simulink model "Mission_Server_Swarm_2QDrone"  (Simulink 9.1)
settings: Solver=ode2  StartTime=0.0  StopTime=inf  FixedStep=0.001  RelTol=1e-3  EnableMultiTasking=on
undefined symbols (not defined in the file): Host, qc_get_step_size
libraries: quarc_library x31, simulink x8
(part 1 of 2)
settings Model: Creator=Admin  LastModifiedBy=jpineros  SimulationMode=external  ExtModeTrigDuration=10000
settings SolverCC: PositivePriorityOrder=on
settings DataIOCC: SaveFormat=Dataset
settings OptimizationCC: LifeSpan=auto
settings DebuggingCC: UnderspecifiedInitializationDetection=Simplified  MergeDetectMultiDrivingBlocksExec=error
settings HardwareCC: ProdBitPerPointer=64  ProdBitPerSizeT=64  ProdBitPerPtrDiffT=64  ProdLargestAtomicFloat=Float  ProdIntDivRoundTo=Zero  ProdEndianess=LittleEndian  ProdWordSize=64  ProdHWDeviceType=Intel->x86-64 (Windows64)
settings ModelReferenceCC: PropagateSignalLabelsOutOfModel=on
settings RTWCC: SystemTargetFile=quarc_win64.tlc  TemplateMakefile=quarc_default_tmf  Description=QUARC Win64 Target Using Toolchain  Toolchain=QUARC win64 | nmake (64-bit Windows)  BuildConfiguration=Faster Runs
settings STFCustomTargetCC: ConcurrentExecutionCompliant=on  UseToolchainInfoCompliant=on  SystemTargetFile=quarc_win64.tlc
settings GRTTargetCC: ParMdlRefBuildCompliant=off  CompOptLevelCompliant=off  MatFileLogging=off  CPPClassGenCompliant=off  ExtMode=on  ExtModeMexFile=quarc_comm
settings ConfigComp: CovHtmlReporting=off

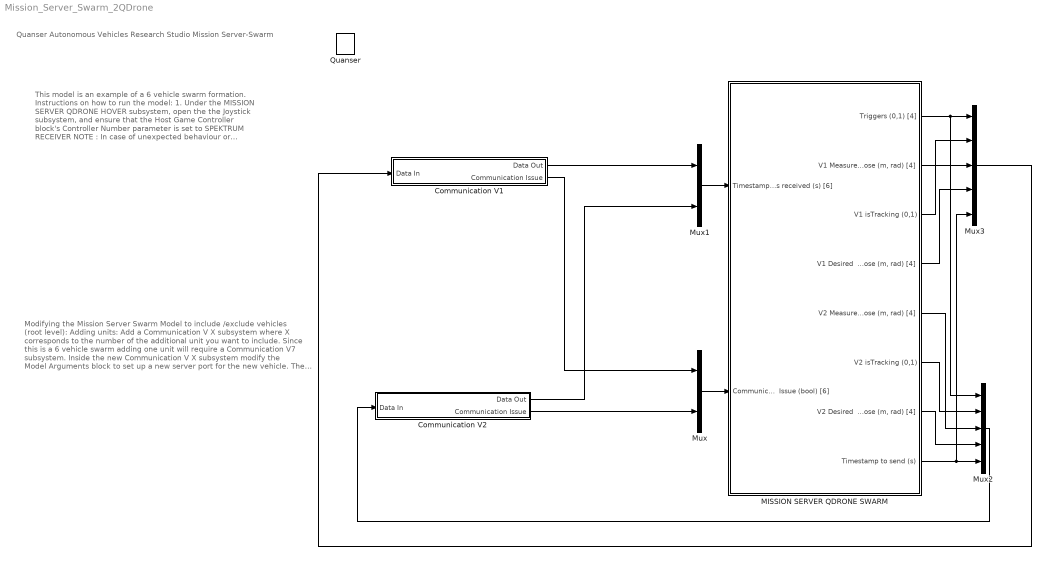
== system Mission_Server_Swarm_2QDrone ==
  note: Modifying the Mission Server Swarm Model to include /exclude vehicles (root level):
      |
      | Adding units:
      | Add a Communication V X subsystem where X corresponds to the number of the additional unit you want to include. Since this is a 6 vehicle swarm adding one unit will require a Communication V7 subsystem.
      | Inside the new Communication V X subsystem modify the Model Arguments block to set up a new server port for the new vehicle. The convention for the Model arguments is URI_Host_V X , where X corresponds to the number of the additional unit you want to include.
      | Go to Simulation\Model Configuration Parameters\Code Generation\Interface in here modify the MEX-File Arguments to include the new Model Argument defined in step 2. This is also where the new port number related to the new vehicle needs to be defined. The format for this new argument should be -URI_Host_VX tcpip://localhost:1800X and must be included within the identifiers ' ' . An example of a modied MEX-Files Arguments string for a 7 vehicle case looks as follows: '-w -d %d -uri %u -URI_Host_V1 tcpip://localhost:18001 -URI_Host_V2 tcpip://localhost:18002 -URI_Host_V3 tcpip://localhost:18003 -URI_Host_V4 tcpip://localhost:18004 -URI_Host_V5 tcpip://localhost:18005 -URI_Host_V6 tcpip://localhost:18006 -URI_Host_V7 tcpip://localhost:18007'
      | Go inside the MISSION SERVER QDRONE SWARM subsystem and follow the instructions on how to add additional units.
      |
      | Removing Units:
      | Remove the excess number of Communication VX subsystems.
      | Go to Simulation\Model Configuration Parameters\Code Generation\Interface in here modify the MEX-File Arguments to match the new number of Communication VX subsystems that you would like to use. An example of a modifified MEX-File Arguments string for a 3 vehicle case looks as follows: '-w -d %d -uri %u -URI_Host_V1 tcpip://localhost:18001 -URI_Host_V2 tcpip://localhost:18002 -URI_Host_V3 tcpip://localhost:18003'
      | Go inside the MISSION SERVER QDRONE SWARM subsystem and follow the instructions on how to remove the number of excess units.
  note: This model is an example of a 6 vehicle swarm formation.
      |
      | Instructions on how to run the model:
      |
      | 1. Under the MISSION SERVER QDRONE HOVER subsystem, open the the Joystick subsystem, and ensure that the Host Game Controller block's Controller Number parameter is set to SPEKTRUM RECEIVER
      | NOTE : In case of unexpected behaviour or emergencies, use the Emergency Abort to cut all power to the motors (this will result in the drone falling). This
      | 2. Configure the localization information for the 6 agents in the Data Server (Localization) subsystem.
      | 3. Under the QUARC menu, click on Build .
      | 4. Under the QUARC menu, click on Start . Wait for the model to start running.
      | 5. Ensure that the isTracking? display shows 1 and that the Joystick Issue display shows 0 (joystick must be powered ON with USB dongle attached to the PC).
      |
      | NOTE : At the start of the model the Comm Issue with Commander display SHOULD display 0. Once the Commander_Stabilizer has successfully connected to the mission server the communication issue flag will update. Landing the QDrones will stop the Commander_Stabilizer model at which point the Comm Issue with Commander should show 1. To close the warning window please stop the Mission_Server_Swarm model.
  note: Quanser Autonomous Vehicles Research Studio
      | Mission Server-Swarm
  Communication V1 : Subsystem
  Communication V2 : Subsystem
  MISSION SERVER QDRONE SWARM : Subsystem
  Mux : Mux  Inputs=2
  Mux1 : Mux  Inputs=2
  Mux2 : Mux  Inputs=5
  Mux3 : Mux  Inputs=5
  Quanser : quarc_library/Logos/Quanser
  wires:
  Mux/1 -> MISSION SERVER QDRONE SWARM/2(Communication  Issue (bool) [6])
  Mux1/1 -> MISSION SERVER QDRONE SWARM/1(Timestamps received (s) [6])
  MISSION SERVER QDRONE SWARM/3(V1 isTracking (0,1)) -> Mux3/2
  MISSION SERVER QDRONE SWARM/1(Triggers (0,1) [4]) -> Mux2/1, Mux3/1
  MISSION SERVER QDRONE SWARM/4("V1 Desired  Pose (m, rad) [4]") -> Mux3/4
  Mux3/1 -> Communication V1/1(Data In)
  Mux2/1 -> Communication V2/1(Data In)
  MISSION SERVER QDRONE SWARM/2("V1 Measured  Pose (m, rad) [4]") -> Mux3/3
  Communication V1/1(Data Out) -> Mux1/1
  Communication V2/1(Data Out) -> Mux1/2
  Communication V1/2(Communication Issue) -> Mux/1
  Communication V2/2(Communication Issue) -> Mux/2
  MISSION SERVER QDRONE SWARM/6(V2 isTracking (0,1)) -> Mux2/2
  MISSION SERVER QDRONE SWARM/8(Timestamp to send (s)) -> Mux3/5, Mux2/5
  MISSION SERVER QDRONE SWARM/7("V2 Desired  Pose (m, rad) [4]") -> Mux2/4
  MISSION SERVER QDRONE SWARM/5("V2 Measured  Pose (m, rad) [4]") -> Mux2/3

== system Mission_Server_Swarm_2QDrone/Communication V1 ==
  Data In : Inport
  Constant : Constant
  Detect Communication loss : Subsystem
  Model Argument : quarc_library/Sources/Signals/Model Argument  argument_name=URI_Host_V1  has_value=on  data_type_mode=Specify via dialog  data_type=char  max_length=80  default_value=0  variable_size=off
      settings: AttributesFormatString=(-%<argument_name>)  SourceProductName=QUARC Targets
  Stream Server : quarc_library/Communications/Basic/Stream Server  uri_source=External input port  uri=tcpip://localhost:18877  apply_uri_to_all_configs=off  send_buffer_size=1460  receive_buffer_size=1460  byte_order=little endian (Intel - LSB first)  optimization=Minimum latency  send_options=Send most recent data  receive_options=Receive most recent data  default_value=zeros(1,1)  sample_time=qc_get_step_size  active=off  implementation=Use blocking I/O in a separate thread  send_fifo_size=1000  receive_fifo_size=1000  send_priority=0  receive_priority=0  send_dimensions=off  receive_dimensions=off  max_dimensions=-1  data_type=Inherited via back propagation  type_expr=BusObject
  "String Display " : quarc_library/Strings/String Display  alignment=center  display_mode=Single line  sample_time=-1  use_new=off
      settings: SourceProductName=QUARC Targets
  Terminator1 : Terminator
  Terminator2 : Terminator
  Data Out : Outport
  Communication Issue : Outport  Port=2
  wires:
  Detect Communication loss/1(Communication Issue (0,1)) -> Communication Issue/1
  Stream Server/1 -> Detect Communication loss/1(State)
  Stream Server/2 -> Detect Communication loss/2(Error)
  Stream Server/4 -> Data Out/1
  Model Argument/1 -> Stream Server/3, "String Display "/1
  Stream Server/5 -> Terminator1/1
  Stream Server/3 -> Terminator2/1
  Data In/1 -> Stream Server/1
  Constant/1 -> Stream Server/2

== system Mission_Server_Swarm_2QDrone/Communication V2 ==
  Data In : Inport
  Constant : Constant
  Detect Communication loss : Subsystem
  Model Argument : quarc_library/Sources/Signals/Model Argument  argument_name=URI_Host_V2  has_value=on  data_type_mode=Specify via dialog  data_type=char  max_length=80  default_value=0  variable_size=off
      settings: AttributesFormatString=(-%<argument_name>)  SourceProductName=QUARC Targets
  Stream Server : quarc_library/Communications/Basic/Stream Server  uri_source=External input port  uri=tcpip://localhost:18877  apply_uri_to_all_configs=off  send_buffer_size=1460  receive_buffer_size=1460  byte_order=little endian (Intel - LSB first)  optimization=Minimum latency  send_options=Send most recent data  receive_options=Receive most recent data  default_value=zeros(1,1)  sample_time=qc_get_step_size  active=off  implementation=Use blocking I/O in a separate thread  send_fifo_size=1000  receive_fifo_size=1000  send_priority=0  receive_priority=0  send_dimensions=off  receive_dimensions=off  max_dimensions=-1  data_type=Inherited via back propagation  type_expr=BusObject
  "String Display " : quarc_library/Strings/String Display  alignment=center  display_mode=Single line  sample_time=-1  use_new=off
      settings: SourceProductName=QUARC Targets
  Terminator1 : Terminator
  Terminator2 : Terminator
  Data Out : Outport
  Communication Issue : Outport  Port=2
  wires:
  Constant/1 -> Stream Server/2
  Data In/1 -> Stream Server/1
  Stream Server/3 -> Terminator2/1
  Stream Server/5 -> Terminator1/1
  Model Argument/1 -> "String Display "/1, Stream Server/3
  Stream Server/4 -> Data Out/1
  Stream Server/2 -> Detect Communication loss/2(Error)
  Stream Server/1 -> Detect Communication loss/1(State)
  Detect Communication loss/1(Communication Issue (0,1)) -> Communication Issue/1

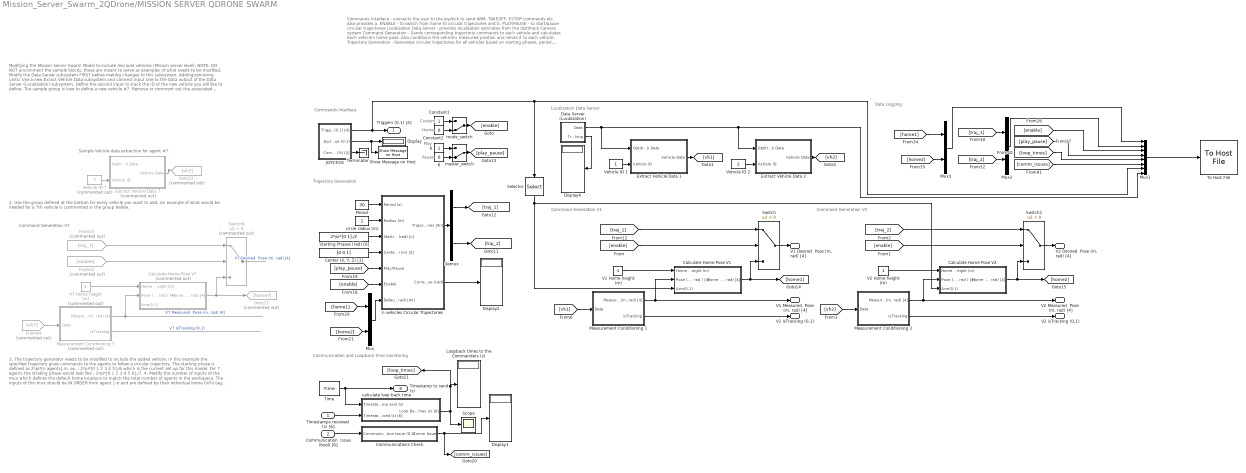
== system Mission_Server_Swarm_2QDrone/MISSION SERVER QDRONE SWARM ==
  note: 3. The trajectory generator needs to be modified to include the added vehicle. In this example
      | the specified trajectory gives commands to the agents to follow a circular trajectory. The starting phase
      | is defined as 2*pi*[n agents]./n, ex. : 2*pi*[0 1 2 3 4 5]./6 which is the current set up for this model. For
      | 7 agents the strating phase would look like : 2*pi*[0 1 2 3 4 5 6]./7.
      |
      | 4. Modify the number of inputs of the mux which defines the default home locations to match the
      | total number of agents in the workspace. The inputs of this mux should be IN ORDER from agent 1-n and
      | are defined by their individual home GoTo tag as seen in the default group commented out in step 7.
      |
      | 5. Adjust the communication and loopback time monitoring logic to add or remove associated
      | sub-blocks as needed.
  note: 2. Use the group defined at the bottom for every vehicle you want to add. An example of what would be needed for a 7th vehicle is commented in the group bellow.
  note: Sample Vehicle data extraction for agent #7.
  note: Modifying the Mission Server Swarm Model to include /exclude vehicles (Mission server level):
      |
      | NOTE: DO NOT uncomment the sample blocks, these are meant to serve as examples of what needs to be modified. Modify the Data Server subsystem FIRST before making changes to this subsystem.
      |
      | Adding\removing units:
      | Use a new Exract Vehicle Data subsystem and connect input one to the Data output of the Data Server (Localization) subsystem. Define the second input to track the ID of the new vehicle you will like to define. The sample group is how to define a new vehicle #7.
      | Remove or comment out the associated subsystem blocks for less number of vehicles.
  note: Commands Interface - connects the user to the joystick to send ARM, TAKEOFF, ESTOP commands etc. Also provides a. ENABLE - to switch from home to circular trajectories and b. PLAY/PAUSE - to start/pause circular trajectories
      | Localization Data Server - provides localization estimates from the Optitrack Camera system
      | Command Generation - Sends corresponding trajectoriy commands to each vehicle and calculates each vehicle's home pose. Also conditions the vehicle's measured position and sends it to each vehicle.
      | Trajectory Generation - Generates circular trajectories for all vehicles based on starting phases, period, radus and center location. When ENABLE is low, it switches to the trajectory at the Default (m, rad) [4] input
      | Communication and Loopback time monitoring - monitors communication issues with any vehicle, and also displays the loopback time to each model (time taken to send a packet to a vehicle and receive it back immediately).
  note: Data Logging
  note: Communication and Loopback time monitoring
  note: Trajectory Generation
  note: Localization Data Server
  note: Commands Interface
  note: Home
  note: Custom
  note: Command Generation V1
  note: Command Generation V2
  note: Pause
  note: Play
  note: Command Generation V7
  Timestamps received (s) [6] : Inport
  Communication  Issue (bool) [6] : Inport  Port=2
  "          6" : Constant
  "   6" : Constant  Value=0
  Calculate Home Pose V1 : Subsystem
  Calculate Home Pose V2 : Subsystem
  Calculate Home Pose V7 : Subsystem  Commented=on
  "Center (X, Y, Z) [3]" : Constant  Value=[0 0 1]
  Communications Check : Subsystem
  Constant2 : Constant  Value=0
  Constant3 : Constant
  "Data Server (Localization) " : Subsystem
  Demux : Demux  Outputs=[4 4]
  Display{,1..2,4} (4 alike) : Display
  Extract Vehicle Data 1 : Subsystem
  Extract Vehicle Data 2 : Subsystem
  Extract Vehicle Data 7 : Subsystem  Commented=on
  From42 : From  Commented=on  GotoTag=enable
  From43 : From  Commented=on  GotoTag=traj_7
  From44 : From  Commented=on  GotoTag=vh7
  Goto22 : Goto  Commented=on  GotoTag=vh7
  Goto23 : Goto  Commented=on  GotoTag=home7
  JOYSTICK : Subsystem
  Loopback times to the Commanders (s) : Display
  Measurement Conditioning 1 : Subsystem
  Measurement Conditioning 2 : Subsystem
  Measurement Conditioning 7 : Subsystem  Commented=on
  Mux : Mux  Inputs=2
  Mux1 : Mux  Inputs=8
  Mux2 : Mux  Inputs=2
  Mux3 : Mux  Inputs=2
  Period : Constant  Value=30
  Scope : Scope
  Selector : Selector  InputPortWidth=4  IndexOptions=Index vector (dialog)  Indices=[1]  OutputSizes=1
  "Show Message on Host " : quarc_library/Sinks/Error Handling/Show Message on Host  message_type=Fixed error message  message_icon=Warning  message=Mission Server: Joystick Disconnected
      settings: AttributesFormatString="\"%<message>\""  SourceProductName=QUARC Targets
  Starting Phases (rad) [6] : Constant  Value=2*pi*[0 1]./2
  Switch : Switch  Criteria=u2 > Threshold
  Switch1 : Switch  Criteria=u2 > Threshold
  Switch6 : Switch  Commented=on  Criteria=u2 > Threshold
  Terminator : Terminator
  Time : quarc_library/Sources/Time/Time  time_source=Wall clock  sample_time=qc_get_step_size
  To Host File : quarc_library/Sinks/To Host/To Host File  file_name=saved_data/%m/%{date}_%{time}.mat  variable_name=data  decimation=1  sample_time=-1  file_format=MAT-file v.4  options=No header or footer  append=off  final_file_name=saved_data/Mission_Server_Swarm_2QDrone/28-Jan-2022_09-46-42.mat  bitrate=2000000
  V1 Home height (m) : Constant
  V2 Home height (m) : Constant
  V7 Home height (m) : Constant  Commented=on
  Vehicle ID 1 : Constant
  "Vehicle ID 2 " : Constant  Value=2
  Vehicle ID 7 : Constant  Commented=on  Value=7
  calculate loop back time : Subsystem
  circle radius (m) : Constant
  master_switch : ManualSwitch  CurrentSetting=0
  mode_switch : ManualSwitch  CurrentSetting=0
  n vehicles Circular Trajectories : Subsystem
  Triggers (0,1) [4] : Outport
  "V1 Measured  Pose (m, rad) [4]" : Outport  Port=2
  V1 isTracking (0,1) : Outport  Port=3
  "V1 Desired  Pose (m, rad) [4]" : Outport  Port=4
  "V2 Measured  Pose (m, rad) [4]" : Outport  Port=5
  V2 isTracking (0,1) : Outport  Port=6
  "V2 Desired  Pose (m, rad) [4]" : Outport  Port=7
  Timestamp to send (s) : Outport  Port=8
  wires:
  JOYSTICK/2(Joystick Issue (0,1)) -> Display/1, "Show Message on Host "/1
  Constant3/1 -> mode_switch/1
  Constant2/1 -> mode_switch/2
  JOYSTICK/3(Commands (%) [4]) -> Terminator/1
  "   6"/1 -> master_switch/2
  Period/1 -> n vehicles Circular Trajectories/1(Period (s))
  circle radius (m)/1 -> n vehicles Circular Trajectories/2(Radius (m))
  "          6"/1 -> master_switch/1
  [play_pause] -> n vehicles Circular Trajectories/5(Play/Pause)
  JOYSTICK/1(Triggers (0,1) [4]) -> Mux1/7, Selector/1, Triggers (0,1) [4]/1
  "Data Server (Localization) "/2(Tracking) -> Display4/1
  Time/1 -> Timestamp to send (s)/1, calculate loop back time/1(Timestamp sent (s))
  Timestamps received (s) [6]/1 -> calculate loop back time/2(Timestamps received (s) [6])
  Starting Phases (rad) [6]/1 -> n vehicles Circular Trajectories/3(Starting Phase (rad) [n])
  "Center (X, Y, Z) [3]"/1 -> n vehicles Circular Trajectories/4(Center (X,Y,Z) (m) [3])
  n vehicles Circular Trajectories/2(Current Phase (rad)) -> Display2/1
  "Vehicle ID 2 "/1 -> Extract Vehicle Data 2/2(Vehicle ID)
  "Data Server (Localization) "/1(Data) -> Extract Vehicle Data 1/1(Optitrack Data), Extract Vehicle Data 2/1(Optitrack Data), Mux1/8
  Vehicle ID 1/1 -> Extract Vehicle Data 1/2(Vehicle ID)
  Measurement Conditioning 1/2(isTracking) -> V1 isTracking (0,1)/1
  Calculate Home Pose V1/1("Home Pose (m, rad) [4]") -> [home1], Switch/3
  [traj_1] -> Switch/1
  V1 Home height (m)/1 -> Calculate Home Pose V1/1(Home height (m))
  Measurement Conditioning 1/1("Measured Pose (m, rad) [4]") -> Calculate Home Pose V1/2("Pose (m, rad ) [4]"), "V1 Measured  Pose (m, rad) [4]"/1
  Switch/1 -> "V1 Desired  Pose (m, rad) [4]"/1
  mode_switch/1 -> [enable]
  [enable] -> Switch/2
  Extract Vehicle Data 1/1(Vehicle Data) -> [vh1]
  Extract Vehicle Data 2/1(Vehicle Data) -> [vh2]
  [vh1] -> Measurement Conditioning 1/1(Data)
  n vehicles Circular Trajectories/1(Trajectories [4n]) -> Demux/1
  Demux/1 -> [traj_1]
  Demux/2 -> [traj_2]
  [vh2] -> Measurement Conditioning 2/1(Data)
  [enable] -> Switch1/2
  Switch1/1 -> "V2 Desired  Pose (m, rad) [4]"/1
  Measurement Conditioning 2/1("Measured Pose (m, rad) [4]") -> Calculate Home Pose V2/2("Pose (m, rad ) [4]"), "V2 Measured  Pose (m, rad) [4]"/1
  V2 Home height (m)/1 -> Calculate Home Pose V2/1(Home height (m))
  [traj_2] -> Switch1/1
  Calculate Home Pose V2/1("Home Pose (m, rad) [4]") -> [home2], Switch1/3
  Measurement Conditioning 2/2(isTracking) -> V2 isTracking (0,1)/1
  [enable] -> n vehicles Circular Trajectories/6(Enable)
  master_switch/1 -> [play_pause]
  Communication  Issue (bool) [6]/1 -> Communications Check/1(Communication Issue (0,1))
  calculate loop back time/1(Loop Back Tmes (s) [6]) -> Scope/1, Loopback times to the Commanders (s)/1, [loop_times]
  Mux/1 -> n vehicles Circular Trajectories/7("Default (m, rad) [4n]")
  [home2] -> Mux/2
  [home1] -> Mux/1
  Mux1/1 -> To Host File/1
  [play_pause] -> Mux1/4
  [enable] -> Mux1/3
  Mux2/1 -> Mux1/2
  [home1] -> Mux3/1
  [home2] -> Mux3/2
  [traj_2] -> Mux2/2
  [traj_1] -> Mux2/1
  Mux3/1 -> Mux1/1
  Communications Check/1(Comm Issue) -> Display1/1, [comm_issues]
  [comm_issues] -> Mux1/6
  [loop_times] -> Mux1/5
  Extract Vehicle Data 7/1(Vehicle Data) -> Goto22/1
  Vehicle ID 7/1 -> Extract Vehicle Data 7/2(Vehicle ID)
  From42/1 -> Switch6/2
  Switch6/1 -> ?  "V7 Desired  Pose (m, rad) [4]"
  From44/1 -> Measurement Conditioning 7/1(Data)
  Measurement Conditioning 7/2(isTracking) -> ?  "V7 isTracking (0,1)"
  From43/1 -> Switch6/1
  V7 Home height (m)/1 -> Calculate Home Pose V7/1(Home height (m))
  Calculate Home Pose V7/1("Home Pose (m, rad) [4]") -> Goto23/1, Switch6/3
  Measurement Conditioning 7/1("Measured Pose (m, rad) [4]") -> Calculate Home Pose V7/2("Pose (m, rad ) [4]")  "V7 Measured  Pose (m, rad) [4]"
  Selector/1 -> Calculate Home Pose V1/3(Arm(0,1)), Calculate Home Pose V2/3(Arm(0,1))
  ? -> Calculate Home Pose V7/3(Arm(0,1))

== system Mission_Server_Swarm_2QDrone/Communication V1/Detect Communication loss ==
  State : Inport
  Error : Inport  Port=2
  Data Type Conversion : DataTypeConversion
  MATLAB Function : MATLAB Function  TreatAsAtomicUnit=on
  Terminator2 : Terminator
  Threshold : quarc_library/Discontinuities/Threshold  operator=>=  param_src=Specify via dialog  threshold=0.5  duration=0.1
      settings: SourceProductName=QUARC Targets
  Time : quarc_library/Sources/Time/Time  time_source=Wall clock  sample_time=qc_get_step_size
  Communication Issue (0,1) : Outport
  wires:
  Threshold/1 -> Data Type Conversion/1
  Data Type Conversion/1 -> Communication Issue (0,1)/1
  Threshold/2 -> Terminator2/1
  Time/1 -> MATLAB Function/1(time)
  State/1 -> MATLAB Function/2(state)
  MATLAB Function/1(stream_connection_loss) -> Threshold/1
  Error/1 -> MATLAB Function/3(error)

== system Mission_Server_Swarm_2QDrone/Communication V2/Detect Communication loss ==
  State : Inport
  Error : Inport  Port=2
  Data Type Conversion : DataTypeConversion
  MATLAB Function : MATLAB Function  TreatAsAtomicUnit=on
  Terminator2 : Terminator
  Threshold : quarc_library/Discontinuities/Threshold  operator=>=  param_src=Specify via dialog  threshold=0.5  duration=0.1
      settings: SourceProductName=QUARC Targets
  Time : quarc_library/Sources/Time/Time  time_source=Wall clock  sample_time=qc_get_step_size
  Communication Issue (0,1) : Outport
  wires:
  Error/1 -> MATLAB Function/3(error)
  MATLAB Function/1(stream_connection_loss) -> Threshold/1
  State/1 -> MATLAB Function/2(state)
  Time/1 -> MATLAB Function/1(time)
  Threshold/2 -> Terminator2/1
  Data Type Conversion/1 -> Communication Issue (0,1)/1
  Threshold/1 -> Data Type Conversion/1

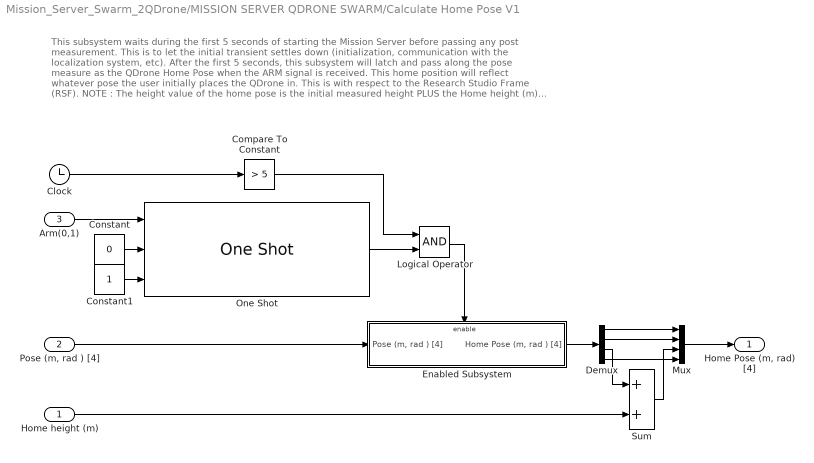
== system Mission_Server_Swarm_2QDrone/MISSION SERVER QDRONE SWARM/Calculate Home Pose V1 ==
  note: This subsystem waits during the first 5 seconds of starting the Mission Server before passing any post measurement.
      | This is to let the initial transient settles down (initialization, communication with the localization system, etc).
      | After the first 5 seconds, this subsystem will latch and pass along the pose measure as the QDrone Home Pose when
      | the ARM signal is received.
      | This home position will reflect whatever pose the user initially places the QDrone in.
      | This is with respect to the Research Studio Frame (RSF).
      |
      | NOTE : The height value of the home pose is the initial measured height PLUS the Home height (m) input value.
  Home height (m) : Inport
  "Pose (m, rad ) [4]" : Inport  Port=2
  Arm(0,1) : Inport  Port=3
  Clock : Clock
  Compare To Constant : simulink/Logic and Bit Operations/Compare To Constant  relop=>  const=5  OutDataTypeStr=boolean
  Constant : Constant  Value=0
  Constant1 : Constant
  Demux : Demux
  Enabled Subsystem : Subsystem  TreatAsAtomicUnit=on
  Logical Operator : Logic  AllPortsSameDT=off  OutDataTypeStr=boolean
  Mux : Mux
  One Shot : quarc_library/Discontinuities/One Shot  trigger_type=Rising edge  redun_pulse=Ignore extraneous pulse  width_source=Specify via dialog  pulse_width=1/qc_get_step_size
      settings: SourceProductName=QUARC Targets
  Sum : Sum
  "Home Pose (m, rad) [4]" : Outport
  wires:
  Constant/1 -> One Shot/2
  Constant1/1 -> One Shot/3
  Arm(0,1)/1 -> One Shot/1
  One Shot/1 -> Logical Operator/2
  "Pose (m, rad ) [4]"/1 -> Enabled Subsystem/1("Pose (m, rad ) [4] ")
  Clock/1 -> Compare To Constant/1
  Compare To Constant/1 -> Logical Operator/1
  Logical Operator/1 -> Enabled Subsystem/Enable
  Enabled Subsystem/1("Home Pose (m, rad ) [4]") -> Demux/1
  Demux/1 -> Mux/1
  Demux/2 -> Mux/2
  Demux/4 -> Mux/4
  Demux/3 -> Sum/1
  Sum/1 -> Mux/3
  Home height (m)/1 -> Sum/2
  Mux/1 -> "Home Pose (m, rad) [4]"/1

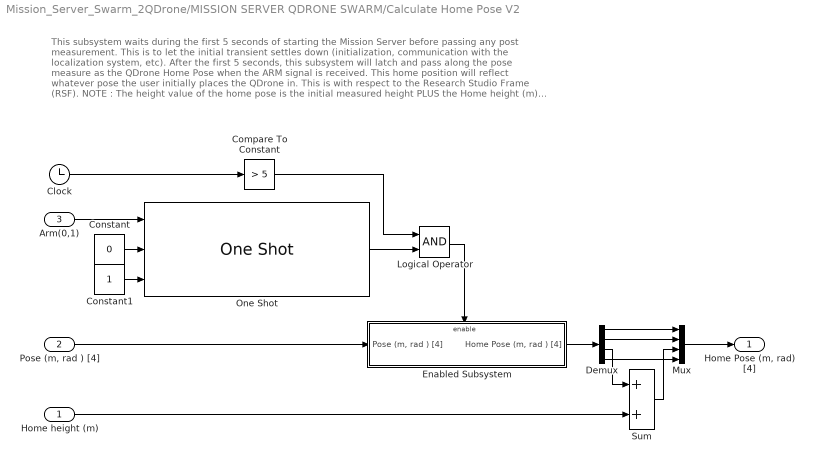
== system Mission_Server_Swarm_2QDrone/MISSION SERVER QDRONE SWARM/Calculate Home Pose V2 ==
  note: This subsystem waits during the first 5 seconds of starting the Mission Server before passing any post measurement.
      | This is to let the initial transient settles down (initialization, communication with the localization system, etc).
      | After the first 5 seconds, this subsystem will latch and pass along the pose measure as the QDrone Home Pose when
      | the ARM signal is received.
      | This home position will reflect whatever pose the user initially places the QDrone in.
      | This is with respect to the Research Studio Frame (RSF).
      |
      | NOTE : The height value of the home pose is the initial measured height PLUS the Home height (m) input value.
  Home height (m) : Inport
  "Pose (m, rad ) [4]" : Inport  Port=2
  Arm(0,1) : Inport  Port=3
  Clock : Clock
  Compare To Constant : simulink/Logic and Bit Operations/Compare To Constant  relop=>  const=5  OutDataTypeStr=boolean
  Constant : Constant  Value=0
  Constant1 : Constant
  Demux : Demux
  Enabled Subsystem : Subsystem  TreatAsAtomicUnit=on
  Logical Operator : Logic  AllPortsSameDT=off  OutDataTypeStr=boolean
  Mux : Mux
  One Shot : quarc_library/Discontinuities/One Shot  trigger_type=Rising edge  redun_pulse=Ignore extraneous pulse  width_source=Specify via dialog  pulse_width=1/qc_get_step_size
      settings: SourceProductName=QUARC Targets
  Sum : Sum
  "Home Pose (m, rad) [4]" : Outport
  wires:
  Constant/1 -> One Shot/2
  Constant1/1 -> One Shot/3
  Arm(0,1)/1 -> One Shot/1
  One Shot/1 -> Logical Operator/2
  "Pose (m, rad ) [4]"/1 -> Enabled Subsystem/1("Pose (m, rad ) [4] ")
  Clock/1 -> Compare To Constant/1
  Compare To Constant/1 -> Logical Operator/1
  Logical Operator/1 -> Enabled Subsystem/Enable
  Enabled Subsystem/1("Home Pose (m, rad ) [4]") -> Demux/1
  Demux/1 -> Mux/1
  Demux/2 -> Mux/2
  Demux/4 -> Mux/4
  Demux/3 -> Sum/1
  Sum/1 -> Mux/3
  Home height (m)/1 -> Sum/2
  Mux/1 -> "Home Pose (m, rad) [4]"/1

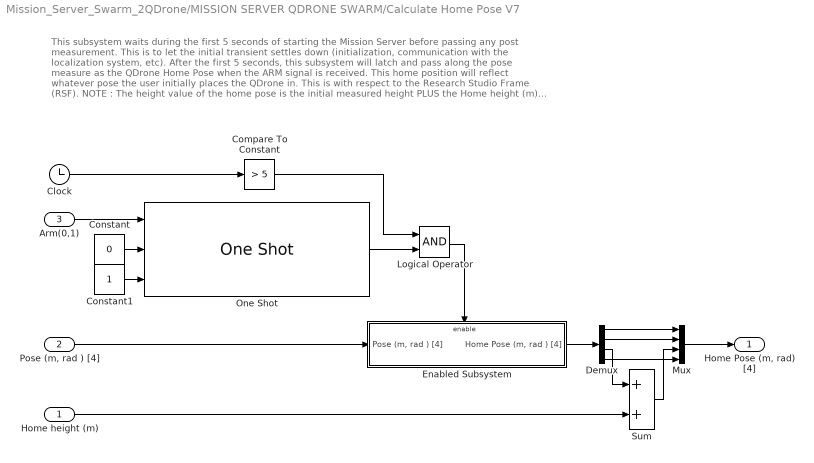
== system Mission_Server_Swarm_2QDrone/MISSION SERVER QDRONE SWARM/Calculate Home Pose V7 ==
  note: This subsystem waits during the first 5 seconds of starting the Mission Server before passing any post measurement.
      | This is to let the initial transient settles down (initialization, communication with the localization system, etc).
      | After the first 5 seconds, this subsystem will latch and pass along the pose measure as the QDrone Home Pose when
      | the ARM signal is received.
      | This home position will reflect whatever pose the user initially places the QDrone in.
      | This is with respect to the Research Studio Frame (RSF).
      |
      | NOTE : The height value of the home pose is the initial measured height PLUS the Home height (m) input value.
  Home height (m) : Inport
  "Pose (m, rad ) [4]" : Inport  Port=2
  Arm(0,1) : Inport  Port=3
  Clock : Clock
  Compare To Constant : simulink/Logic and Bit Operations/Compare To Constant  relop=>  const=5  OutDataTypeStr=boolean
  Constant : Constant  Value=0
  Constant1 : Constant
  Demux : Demux
  Enabled Subsystem : Subsystem  TreatAsAtomicUnit=on
  Logical Operator : Logic  AllPortsSameDT=off  OutDataTypeStr=boolean
  Mux : Mux
  One Shot : quarc_library/Discontinuities/One Shot  trigger_type=Rising edge  redun_pulse=Ignore extraneous pulse  width_source=Specify via dialog  pulse_width=1/qc_get_step_size
      settings: SourceProductName=QUARC Targets
  Sum : Sum
  "Home Pose (m, rad) [4]" : Outport
  wires:
  Constant/1 -> One Shot/2
  Constant1/1 -> One Shot/3
  Arm(0,1)/1 -> One Shot/1
  One Shot/1 -> Logical Operator/2
  "Pose (m, rad ) [4]"/1 -> Enabled Subsystem/1("Pose (m, rad ) [4] ")
  Clock/1 -> Compare To Constant/1
  Compare To Constant/1 -> Logical Operator/1
  Logical Operator/1 -> Enabled Subsystem/Enable
  Enabled Subsystem/1("Home Pose (m, rad ) [4]") -> Demux/1
  Demux/1 -> Mux/1
  Demux/2 -> Mux/2
  Demux/4 -> Mux/4
  Demux/3 -> Sum/1
  Sum/1 -> Mux/3
  Home height (m)/1 -> Sum/2
  Mux/1 -> "Home Pose (m, rad) [4]"/1

== system Mission_Server_Swarm_2QDrone/MISSION SERVER QDRONE SWARM/Communications Check ==
  note: Pass along the communication issue flag only after the connection with the vehicle model was established.
  Communication Issue (0,1) : Inport
  Demux : Demux  Outputs=2
  Logical Operator : Logic  Operator=OR  Inputs=1  AllPortsSameDT=off  OutDataTypeStr=boolean
  Mux : Mux  Inputs=2
  Product : Product
  Product1 : Product
  Show Message on Host : quarc_library/Sinks/Error Handling/Show Message on Host  message_type=Fixed error message  message_icon=Warning  message=Mission Server: Communication Issue with a QDrone
      settings: AttributesFormatString="\"%<message>\""  SourceProductName=QUARC Targets
  Triggered Subsystem : Subsystem  TreatAsAtomicUnit=on
  Triggered Subsystem1 : Subsystem  TreatAsAtomicUnit=on
  Comm Issue : Outport
  wires:
  Communication Issue (0,1)/1 -> Demux/1
  Demux/1 -> Product/1, Triggered Subsystem/Trigger
  Demux/2 -> Product1/1, Triggered Subsystem1/Trigger
  Triggered Subsystem/1(Communication Issue (0,1)) -> Product/2
  Product/1 -> Mux/1
  Mux/1 -> Comm Issue/1, Logical Operator/1
  Logical Operator/1 -> Show Message on Host/1
  Triggered Subsystem1/1(Communication Issue (0,1)) -> Product1/2
  Product1/1 -> Mux/2

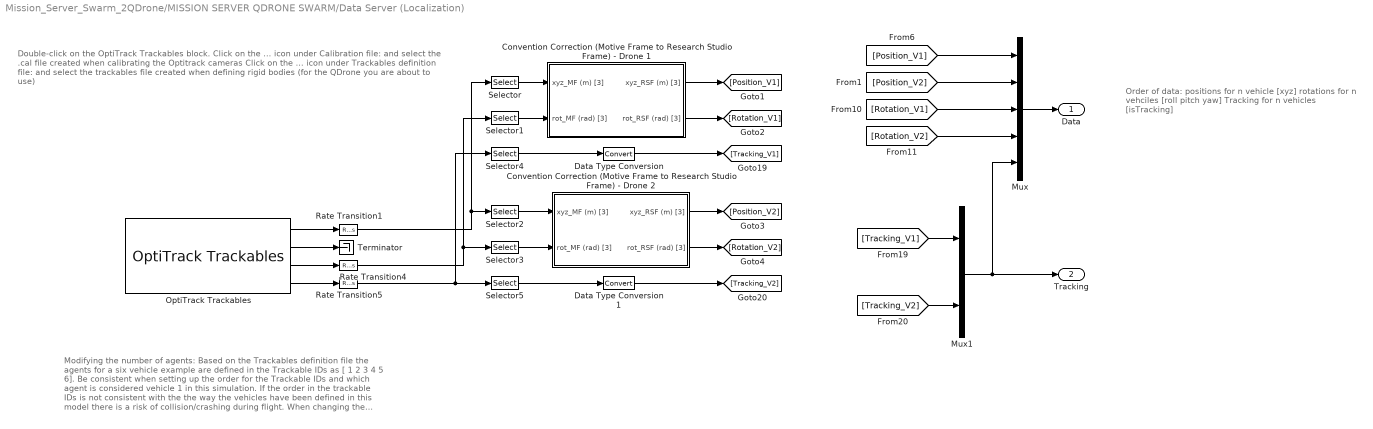
== system Mission_Server_Swarm_2QDrone/MISSION SERVER QDRONE SWARM/Data Server (Localization)  ==
  note: Order of data:
      |
      | positions for n vehicle [xyz]
      | rotations for n vehciles [roll pitch yaw]
      | Tracking for n vehicles [isTracking]
  note: Modifying the number of agents:
      |
      | Based on the Trackables definition file the agents for a six vehicle example are defined in the Trackable IDs as [ 1 2 3 4 5 6]. Be consistent when setting up the order for the Trackable IDs and which agent is considered vehicle 1 in this simulation. If the order in the trackable IDs is not consistent with the the way the vehicles have been defined in this model there is a risk of collision/crashing during flight.
      | When changing the number of agents please update the selectors which are used to parase the data going into the individual Convention Correction subsystem. The RED selectors have signal dimension 3*n (where n is the number of vehicles). The YELLOW selectors have signal dimension n.
  note: Double-click on the OptiTrack Trackables block.
      |
      | Click on the ... icon under Calibration file: and select the .cal file
      | created when calibrating the Optitrack cameras
      |
      | Click on the ... icon under Trackables definition file: and select
      | the trackables file created when defining rigid bodies (for the
      | QDrone you are about to use)
  Convention Correction (Motive Frame to Research Studio Frame) - Drone 1 : Subsystem
  Convention Correction (Motive Frame to Research Studio Frame) - Drone 2 : Subsystem
  Data Type Conversion : DataTypeConversion
  Data Type Conversion1 : DataTypeConversion
  Mux : Mux  Inputs=5
  Mux1 : Mux  Inputs=2
  OptiTrack Trackables : quarc_library/Devices/Third-Party/NaturalPoint/OptiTrack/OptiTrack Trackables  calibration_file=C:\Users\user\Documents\optitrack\180825\Calibration Exceptional (MeanErr 0.613 mm) 2018-08-25 12.58pm.cal  rigid_body_file=C:\Users\user\Documents\optitrack\180825\qdrone_1.tra  rigid_body_ids=[1 2 ]  sample_time=qc_get_step_size*10  active=off
      settings: SourceProductName=QUARC Targets
  Rate Transition1 : RateTransition
  Rate Transition4 : RateTransition
  Rate Transition5 : RateTransition
  Selector : Selector  InputPortWidth=6  IndexOptions=Index vector (dialog)  Indices=[1:3]  OutputSizes=1
  Selector1 : Selector  InputPortWidth=6  IndexOptions=Index vector (dialog)  Indices=[1:3]  OutputSizes=1
  Selector2 : Selector  InputPortWidth=6  IndexOptions=Index vector (dialog)  Indices=[4:6]  OutputSizes=1
  Selector3 : Selector  InputPortWidth=6  IndexOptions=Index vector (dialog)  Indices=[4:6]  OutputSizes=1
  Selector4 : Selector  InputPortWidth=2  IndexOptions=Index vector (dialog)  Indices=[1]  OutputSizes=1
  Selector5 : Selector  InputPortWidth=2  IndexOptions=Index vector (dialog)  Indices=[2]  OutputSizes=1
  Terminator : Terminator
  Data : Outport
  Tracking : Outport  Port=2
  wires:
  OptiTrack Trackables/4 -> Rate Transition5/1
  OptiTrack Trackables/1 -> Rate Transition1/1
  OptiTrack Trackables/3 -> Rate Transition4/1
  Rate Transition4/1 -> Selector1/1, Selector3/1
  Convention Correction (Motive Frame to Research Studio Frame) - Drone 2/2(rot_RSF (rad) [3]) -> [Rotation_V2]
  Selector1/1 -> Convention Correction (Motive Frame to Research Studio Frame) - Drone 1/2(rot_MF (rad) [3])
  Rate Transition5/1 -> Selector4/1, Selector5/1
  Data Type Conversion/1 -> [Tracking_V1]
  Selector/1 -> Convention Correction (Motive Frame to Research Studio Frame) - Drone 1/1(xyz_MF (m) [3])
  Convention Correction (Motive Frame to Research Studio Frame) - Drone 2/1(xyz_RSF (m) [3]) -> [Position_V2]
  Convention Correction (Motive Frame to Research Studio Frame) - Drone 1/1(xyz_RSF (m) [3]) -> [Position_V1]
  OptiTrack Trackables/2 -> Terminator/1
  Selector5/1 -> Data Type Conversion1/1
  Convention Correction (Motive Frame to Research Studio Frame) - Drone 1/2(rot_RSF (rad) [3]) -> [Rotation_V1]
  Selector4/1 -> Data Type Conversion/1
  Selector3/1 -> Convention Correction (Motive Frame to Research Studio Frame) - Drone 2/2(rot_MF (rad) [3])
  Data Type Conversion1/1 -> [Tracking_V2]
  Selector2/1 -> Convention Correction (Motive Frame to Research Studio Frame) - Drone 2/1(xyz_MF (m) [3])
  Rate Transition1/1 -> Selector/1, Selector2/1
  [Position_V2] -> Mux/2
  [Tracking_V1] -> Mux1/1
  [Rotation_V1] -> Mux/3
  [Position_V1] -> Mux/1
  [Tracking_V2] -> Mux1/2
  [Rotation_V2] -> Mux/4
  Mux1/1 -> Mux/5, Tracking/1
  Mux/1 -> Data/1

== system Mission_Server_Swarm_2QDrone/MISSION SERVER QDRONE SWARM/Extract Vehicle Data 1 ==
  Optitrack Data : Inport
  Vehicle ID : Inport  Port=2
  Data Type Conversion10 : DataTypeConversion
  Data Type Conversion11 : DataTypeConversion
  Data Type Conversion9 : DataTypeConversion
  Extract Object Data : MATLAB Function  TreatAsAtomicUnit=on
  Mux1 : Mux  Inputs=3
  Reshape : Reshape
  Reshape1 : Reshape
  Reshape2 : Reshape
  Vehicle Data : Outport
  wires:
  Reshape2/1 -> Data Type Conversion9/1
  Reshape1/1 -> Data Type Conversion10/1
  Reshape/1 -> Data Type Conversion11/1
  Data Type Conversion9/1 -> Mux1/3
  Data Type Conversion10/1 -> Mux1/2
  Data Type Conversion11/1 -> Mux1/1
  Extract Object Data/2(orientation) -> Reshape1/1
  Extract Object Data/3(tracking) -> Reshape2/1
  Extract Object Data/1(position) -> Reshape/1
  Mux1/1 -> Vehicle Data/1
  Optitrack Data/1 -> Extract Object Data/1(data)
  Vehicle ID/1 -> Extract Object Data/2(index)

== system Mission_Server_Swarm_2QDrone/MISSION SERVER QDRONE SWARM/Extract Vehicle Data 2 ==
  Optitrack Data : Inport
  Vehicle ID : Inport  Port=2
  Data Type Conversion10 : DataTypeConversion
  Data Type Conversion11 : DataTypeConversion
  Data Type Conversion9 : DataTypeConversion
  Extract Object Data : MATLAB Function  TreatAsAtomicUnit=on
  Mux1 : Mux  Inputs=3
  Reshape : Reshape
  Reshape1 : Reshape
  Reshape2 : Reshape
  Vehicle Data : Outport
  wires:
  Vehicle ID/1 -> Extract Object Data/2(index)
  Optitrack Data/1 -> Extract Object Data/1(data)
  Mux1/1 -> Vehicle Data/1
  Extract Object Data/1(position) -> Reshape/1
  Extract Object Data/3(tracking) -> Reshape2/1
  Extract Object Data/2(orientation) -> Reshape1/1
  Data Type Conversion11/1 -> Mux1/1
  Data Type Conversion10/1 -> Mux1/2
  Data Type Conversion9/1 -> Mux1/3
  Reshape/1 -> Data Type Conversion11/1
  Reshape1/1 -> Data Type Conversion10/1
  Reshape2/1 -> Data Type Conversion9/1

== system Mission_Server_Swarm_2QDrone/MISSION SERVER QDRONE SWARM/Extract Vehicle Data 7 ==
  Optitrack Data : Inport
  Vehicle ID : Inport  Port=2
  Data Type Conversion10 : DataTypeConversion
  Data Type Conversion11 : DataTypeConversion
  Data Type Conversion9 : DataTypeConversion
  Extract Object Data : MATLAB Function  TreatAsAtomicUnit=on
  Mux1 : Mux  Inputs=3
  Reshape : Reshape
  Reshape1 : Reshape
  Reshape2 : Reshape
  Vehicle Data : Outport
  wires:
  Reshape2/1 -> Data Type Conversion9/1
  Reshape1/1 -> Data Type Conversion10/1
  Reshape/1 -> Data Type Conversion11/1
  Data Type Conversion9/1 -> Mux1/3
  Data Type Conversion10/1 -> Mux1/2
  Data Type Conversion11/1 -> Mux1/1
  Extract Object Data/2(orientation) -> Reshape1/1
  Extract Object Data/3(tracking) -> Reshape2/1
  Extract Object Data/1(position) -> Reshape/1
  Mux1/1 -> Vehicle Data/1
  Optitrack Data/1 -> Extract Object Data/1(data)
  Vehicle ID/1 -> Extract Object Data/2(index)

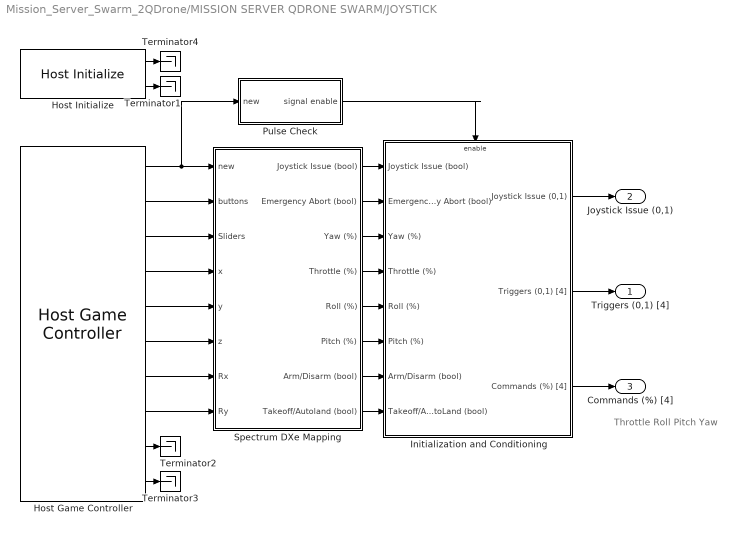
== system Mission_Server_Swarm_2QDrone/MISSION SERVER QDRONE SWARM/JOYSTICK ==
  note: Throttle
      | Roll
      | Pitch
      | Yaw
  Host Game Controller : quarc_library/Devices/Peripherals/Host/Host Game Controller  object_name=Host-1  controller=1  buffer_size=20  deadzone=[]  saturation=[]  sample_time=qc_get_step_size  auto_center=off  enabled=on  debug_mode=off
      settings: SourceProductName=QUARC Targets
  Host Initialize : quarc_library/Devices/Peripherals/Host/Host Initialize  object_name=Host-1  uri_source=Use external mode communications  uri=tcpip://localhost:18001  apply_uri_to_all_configs=on  send_buffer_size=1000  receive_buffer_size=1000  thread_priority=0  run_client=on  use_window=off  window_position=[]  sample_time=qc_get_step_size  active=on
      settings: SourceProductName=QUARC Targets
  Initialization and Conditioning : Subsystem  TreatAsAtomicUnit=on
  Pulse Check : Subsystem  TreatAsAtomicUnit=on
  Spectrum DXe Mapping : Subsystem
  Terminator{1..4} (4 alike) : Terminator
  Triggers (0,1) [4] : Outport
  Joystick Issue (0,1) : Outport  Port=2
  Commands (%) [4] : Outport  Port=3
  wires:
  Pulse Check/1(signal enable) -> Initialization and Conditioning/Enable
  Host Game Controller/1 -> Pulse Check/1(new), Spectrum DXe Mapping/1(new)
  Initialization and Conditioning/3(Commands (%) [4]) -> Commands (%) [4]/1
  Spectrum DXe Mapping/8(Takeoff/Autoland (bool)) -> Initialization and Conditioning/8(Takeoff/AutoLand (bool))
  Initialization and Conditioning/2(Triggers (0,1) [4]) -> Triggers (0,1) [4]/1
  Spectrum DXe Mapping/2(Emergency Abort (bool)) -> Initialization and Conditioning/2(Emergency Abort (bool))
  Host Game Controller/2 -> Spectrum DXe Mapping/2(buttons)
  Spectrum DXe Mapping/6(Pitch (%)) -> Initialization and Conditioning/6(Pitch (%))
  Spectrum DXe Mapping/4(Throttle (%)) -> Initialization and Conditioning/4(Throttle (%))
  Spectrum DXe Mapping/5(Roll (%)) -> Initialization and Conditioning/5(Roll (%))
  Spectrum DXe Mapping/7("Arm/Disarm (bool) ") -> Initialization and Conditioning/7(Arm/Disarm (bool))
  Spectrum DXe Mapping/3(Yaw (%)) -> Initialization and Conditioning/3(Yaw (%))
  Host Initialize/2 -> Terminator1/1
  Host Initialize/1 -> Terminator4/1
  Host Game Controller/6 -> Spectrum DXe Mapping/6(z)
  Host Game Controller/3 -> Spectrum DXe Mapping/3(Sliders)
  Host Game Controller/5 -> Spectrum DXe Mapping/5(y)
  Host Game Controller/4 -> Spectrum DXe Mapping/4(x)
  Host Game Controller/8 -> Spectrum DXe Mapping/8(Ry)
  Host Game Controller/9 -> Terminator2/1
  Host Game Controller/10 -> Terminator3/1
  Host Game Controller/7 -> Spectrum DXe Mapping/7(Rx)
  Spectrum DXe Mapping/1(Joystick Issue (bool)) -> Initialization and Conditioning/1(Joystick Issue (bool))
  Initialization and Conditioning/1(Joystick Issue (0,1)) -> Joystick Issue (0,1)/1

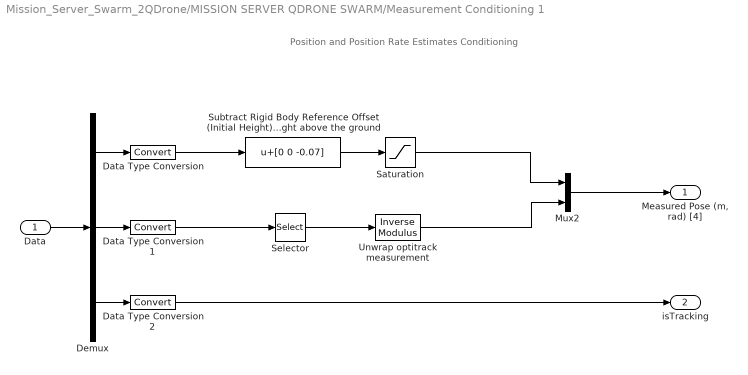
== system Mission_Server_Swarm_2QDrone/MISSION SERVER QDRONE SWARM/Measurement Conditioning 1 ==
  note: Position and Position Rate Estimates Conditioning
  Data : Inport
  Data Type Conversion : DataTypeConversion
  Data Type Conversion1 : DataTypeConversion
  Data Type Conversion2 : DataTypeConversion
  Demux : Demux  Outputs=[3 3 1]
  Mux2 : Mux  Inputs=[3 1]
  Saturation : Saturate  UpperLimit=[2 2 3]  LowerLimit=[-2 -2 0]
  Selector : Selector  InputPortWidth=3  IndexOptions=Index vector (dialog)  Indices=[3]  OutputSizes=1
  Subtract Rigid Body Reference Offset (Initial Height)  to get height above the ground : Bias  Bias=[0 0 -0.07]
  Unwrap optitrack measurement : quarc_library/Discontinuities/Inverse Modulus  modulus=2*pi  output_derivative=off  output_revolutions=off  max_x=Inf  min_x=-Inf
  "Measured Pose (m, rad) [4]" : Outport
  isTracking : Outport  Port=2
  wires:
  Demux/2 -> Data Type Conversion1/1
  Demux/1 -> Data Type Conversion/1
  Demux/3 -> Data Type Conversion2/1
  Mux2/1 -> "Measured Pose (m, rad) [4]"/1
  Data/1 -> Demux/1
  Data Type Conversion2/1 -> isTracking/1
  Subtract Rigid Body Reference Offset (Initial Height)  to get height above the ground/1 -> Saturation/1
  Saturation/1 -> Mux2/1
  Data Type Conversion1/1 -> Selector/1
  Selector/1 -> Unwrap optitrack measurement/1
  Data Type Conversion/1 -> Subtract Rigid Body Reference Offset (Initial Height)  to get height above the ground/1
  Unwrap optitrack measurement/1 -> Mux2/2

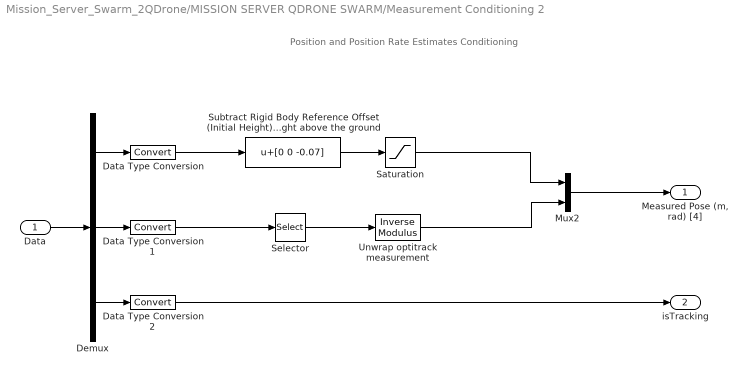
== system Mission_Server_Swarm_2QDrone/MISSION SERVER QDRONE SWARM/Measurement Conditioning 2 ==
  note: Position and Position Rate Estimates Conditioning
  Data : Inport
  Data Type Conversion : DataTypeConversion
  Data Type Conversion1 : DataTypeConversion
  Data Type Conversion2 : DataTypeConversion
  Demux : Demux  Outputs=[3 3 1]
  Mux2 : Mux  Inputs=[3 1]
  Saturation : Saturate  UpperLimit=[2 2 3]  LowerLimit=[-2 -2 0]
  Selector : Selector  InputPortWidth=3  IndexOptions=Index vector (dialog)  Indices=[3]  OutputSizes=1
  Subtract Rigid Body Reference Offset (Initial Height)  to get height above the ground : Bias  Bias=[0 0 -0.07]
  Unwrap optitrack measurement : quarc_library/Discontinuities/Inverse Modulus  modulus=2*pi  output_derivative=off  output_revolutions=off  max_x=Inf  min_x=-Inf
  "Measured Pose (m, rad) [4]" : Outport
  isTracking : Outport  Port=2
  wires:
  Demux/2 -> Data Type Conversion1/1
  Demux/1 -> Data Type Conversion/1
  Demux/3 -> Data Type Conversion2/1
  Mux2/1 -> "Measured Pose (m, rad) [4]"/1
  Data/1 -> Demux/1
  Data Type Conversion2/1 -> isTracking/1
  Subtract Rigid Body Reference Offset (Initial Height)  to get height above the ground/1 -> Saturation/1
  Saturation/1 -> Mux2/1
  Data Type Conversion1/1 -> Selector/1
  Selector/1 -> Unwrap optitrack measurement/1
  Data Type Conversion/1 -> Subtract Rigid Body Reference Offset (Initial Height)  to get height above the ground/1
  Unwrap optitrack measurement/1 -> Mux2/2

== system Mission_Server_Swarm_2QDrone/MISSION SERVER QDRONE SWARM/Measurement Conditioning 7 ==
  note: Position and Position Rate Estimates Conditioning
  Data : Inport
  Data Type Conversion : DataTypeConversion
  Data Type Conversion1 : DataTypeConversion
  Data Type Conversion2 : DataTypeConversion
  Demux : Demux  Outputs=[3 3 1]
  Mux2 : Mux  Inputs=[3 1]
  Saturation : Saturate  UpperLimit=[2 2 3]  LowerLimit=[-2 -2 0]
  Selector : Selector  InputPortWidth=3  IndexOptions=Index vector (dialog)  Indices=[3]  OutputSizes=1
  Subtract Rigid Body Reference Offset (Initial Height)  to get height above the ground : Bias  Bias=[0 0 -0.07]
  Unwrap optitrack measurement : quarc_library/Discontinuities/Inverse Modulus  modulus=2*pi  output_derivative=off  output_revolutions=off  max_x=Inf  min_x=-Inf
  "Measured Pose (m, rad) [4]" : Outport
  isTracking : Outport  Port=2
  wires:
  Demux/2 -> Data Type Conversion1/1
  Demux/1 -> Data Type Conversion/1
  Demux/3 -> Data Type Conversion2/1
  Mux2/1 -> "Measured Pose (m, rad) [4]"/1
  Data/1 -> Demux/1
  Data Type Conversion2/1 -> isTracking/1
  Subtract Rigid Body Reference Offset (Initial Height)  to get height above the ground/1 -> Saturation/1
  Saturation/1 -> Mux2/1
  Data Type Conversion1/1 -> Selector/1
  Selector/1 -> Unwrap optitrack measurement/1
  Data Type Conversion/1 -> Subtract Rigid Body Reference Offset (Initial Height)  to get height above the ground/1
  Unwrap optitrack measurement/1 -> Mux2/2

== system Mission_Server_Swarm_2QDrone/MISSION SERVER QDRONE SWARM/calculate loop back time ==
  Timestamp sent (s) : Inport
  Timestamps received (s) [6] : Inport  Port=2
  Demux : Demux  Outputs=2
  Mux : Mux  Inputs=2
  Subtract : Sum  Inputs=+-
  Subtract1 : Sum  Inputs=+-
  Loop Back Tmes (s) [6] : Outport
  wires:
  Timestamp sent (s)/1 -> Subtract1/1, Subtract/1
  Timestamps received (s) [6]/1 -> Demux/1
  Demux/1 -> Subtract/2
  Demux/2 -> Subtract1/2
  Subtract/1 -> Mux/1
  Subtract1/1 -> Mux/2
  Mux/1 -> Loop Back Tmes (s) [6]/1

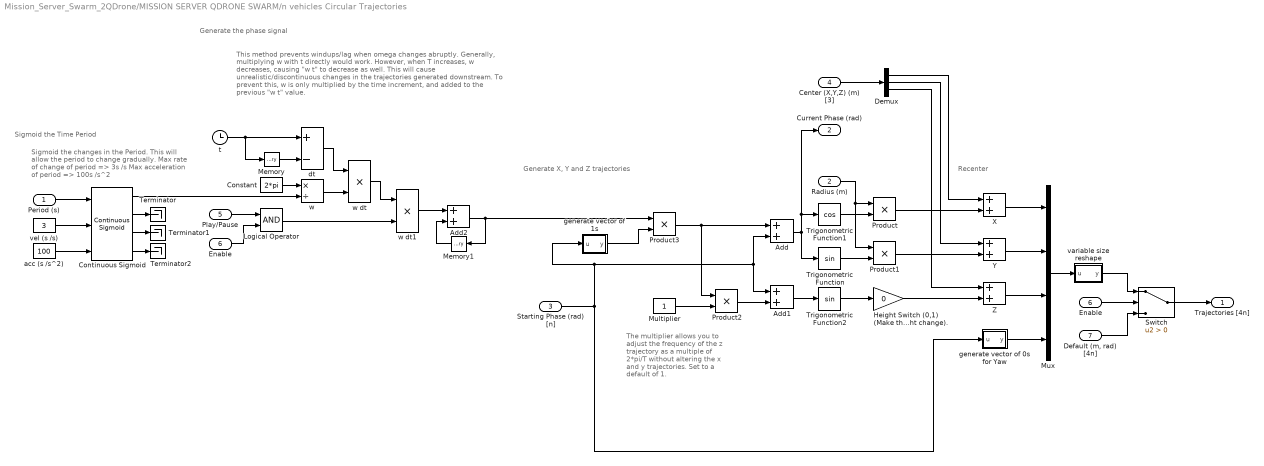
== system Mission_Server_Swarm_2QDrone/MISSION SERVER QDRONE SWARM/n vehicles Circular Trajectories ==
  note: Recenter
  note: Generate X, Y and Z trajectories
  note: Generate the phase signal
  note: Sigmoid the changes in the Period. This will
      | allow the period to change gradually.
      | Max rate of change of period => 3s /s
      | Max acceleration of period => 100s /s^2
  note: Sigmoid the Time Period
  note: The multiplier allows you to adjust the frequency of the z trajectory as a multiple of 2*pi/T without altering the x and y trajectories. Set to a default of 1.
  note: This method prevents windups/lag when omega changes abruptly. Generally, multiplying w with t directly would work. However, when T increases, w decreases, causing "w t" to decrease as well. This will cause unrealistic/discontinuous changes in the trajectories generated downstream.
      |
      | To prevent this, w is only multiplied by the time increment, and added to the previous "w t" value.
  Period (s) : Inport
  Radius (m) : Inport  Port=2
  Starting Phase (rad) [n] : Inport  Port=3
  Center (X,Y,Z) (m) [3] : Inport  Port=4
  Play/Pause : Inport  Port=5
  Enable : Inport  Port=6
  "Default (m, rad) [4n]" : Inport  Port=7
  " Enable " : InportShadow  Port=6
  Add : Sum
  Add1 : Sum
  Add2 : Sum
  Constant : Constant  Value=2*pi
  Continuous Sigmoid : quarc_library/Sources/Sigmoids/Continuous Sigmoid  params_source=External (input ports)  max_velocity=2  max_acceleration=10  initial_position=10  initial_velocity=0  hold_off=0.5  input_sample_time=-1  output_sample_time=qc_get_step_size
      settings: SourceProductName=QUARC Targets
  Demux : Demux  Outputs=3
  Height Switch (0,1) (Make this 0 to disable height change). : Gain  Gain=0
  Logical Operator : Logic  AllPortsSameDT=off  OutDataTypeStr=boolean
  Memory : Memory
  Memory1 : Memory
  Multiplier : Constant
  Mux : Mux
  Product{,1..3} (4 alike) : Product
  Switch : Switch  Criteria=u2 > Threshold
  Terminator : Terminator
  Terminator1 : Terminator
  Terminator2 : Terminator
  Trigonometric Function : Trigonometry
  Trigonometric Function1 : Trigonometry  Operator=cos
  Trigonometric Function2 : Trigonometry
  X : Sum
  Y : Sum
  Z : Sum
  acc (s /s^2) : Constant  Value=100
  dt : Sum  Inputs=+-
  generate vector of 0s for Yaw : MATLAB Function  TreatAsAtomicUnit=on
  generate vector of 1s : MATLAB Function  TreatAsAtomicUnit=on
  t : Clock
  variable size reshape : MATLAB Function  TreatAsAtomicUnit=on
  vel (s /s) : Constant  Value=3
  w : Product  Inputs=*/
  w dt : Product
  w dt1 : Product
  Trajectories [4n] : Outport
  Current Phase (rad) : Outport  Port=2
  wires:
  Trigonometric Function/1 -> Product1/2
  Trigonometric Function1/1 -> Product/2
  Height Switch (0,1) (Make this 0 to disable height change)./1 -> Z/2
  Product1/1 -> Y/2
  Product/1 -> X/2
  Radius (m)/1 -> Product/1, Product1/1
  generate vector of 0s for Yaw/1(y) -> Mux/4
  Continuous Sigmoid/4 -> Terminator2/1
  Period (s)/1 -> Continuous Sigmoid/1
  Continuous Sigmoid/2 -> Terminator/1
  Continuous Sigmoid/3 -> Terminator1/1
  acc (s /s^2)/1 -> Continuous Sigmoid/3
  vel (s /s)/1 -> Continuous Sigmoid/2
  Add1/1 -> Trigonometric Function2/1
  Multiplier/1 -> Product2/2
  Starting Phase (rad) [n]/1 -> generate vector of 1s/1(u), Add/2, Add1/1, generate vector of 0s for Yaw/1(u)
  Add2/1 -> Product3/1, Memory1/1
  Add/1 -> Current Phase (rad)/1, Trigonometric Function1/1, Trigonometric Function/1
  Center (X,Y,Z) (m) [3]/1 -> Demux/1
  Demux/2 -> Y/1
  Demux/1 -> X/1
  Trigonometric Function2/1 -> Height Switch (0,1) (Make this 0 to disable height change)./1
  Demux/3 -> Z/1
  X/1 -> Mux/1
  Y/1 -> Mux/2
  Z/1 -> Mux/3
  Memory/1 -> dt/2
  w dt/1 -> w dt1/1
  w dt1/1 -> Add2/1
  Constant/1 -> w/1
  Memory1/1 -> Add2/2
  w/1 -> w dt/2
  Continuous Sigmoid/1 -> w/2
  t/1 -> Memory/1, dt/1
  dt/1 -> w dt/1
  Mux/1 -> variable size reshape/1(u)
  Switch/1 -> Trajectories [4n]/1
  "Default (m, rad) [4n]"/1 -> Switch/3
  Enable/1 -> Switch/2
  Play/Pause/1 -> Logical Operator/1
  " Enable "/1 -> Logical Operator/2
  Logical Operator/1 -> w dt1/2
  Product3/1 -> Add/1, Product2/1
  variable size reshape/1(y) -> Switch/1
  generate vector of 1s/1(y) -> Product3/2
  Product2/1 -> Add1/2

== system Mission_Server_Swarm_2QDrone/MISSION SERVER QDRONE SWARM/Calculate Home Pose V1/Enabled Subsystem ==
  "Pose (m, rad ) [4] " : Inport
  Enable : EnablePort
  "Home Pose (m, rad ) [4]" : Outport
  wires:
  "Pose (m, rad ) [4] "/1 -> "Home Pose (m, rad ) [4]"/1

== system Mission_Server_Swarm_2QDrone/MISSION SERVER QDRONE SWARM/Calculate Home Pose V2/Enabled Subsystem ==
  "Pose (m, rad ) [4] " : Inport
  Enable : EnablePort
  "Home Pose (m, rad ) [4]" : Outport
  wires:
  "Pose (m, rad ) [4] "/1 -> "Home Pose (m, rad ) [4]"/1

== system Mission_Server_Swarm_2QDrone/MISSION SERVER QDRONE SWARM/Calculate Home Pose V7/Enabled Subsystem ==
  "Pose (m, rad ) [4] " : Inport
  Enable : EnablePort
  "Home Pose (m, rad ) [4]" : Outport
  wires:
  "Pose (m, rad ) [4] "/1 -> "Home Pose (m, rad ) [4]"/1

== system Mission_Server_Swarm_2QDrone/MISSION SERVER QDRONE SWARM/Communications Check/Triggered Subsystem ==
  note: This looks for the first falling edge to trigger a communication issue,
      | because the mission server model starts first.
  Trigger : TriggerPort  TriggerType=falling  VariantControl=Variant
  Add : Sum
  Compare To Constant : simulink/Logic and Bit Operations/Compare To Constant  relop=>=  const=1  OutDataTypeStr=boolean
  Constant : Constant
  Memory : Memory  InheritSampleTime=on
  Communication Issue (0,1) : Outport  InitialOutput=0
  wires:
  Constant/1 -> Add/1
  Memory/1 -> Add/2
  Add/1 -> Compare To Constant/1, Memory/1
  Compare To Constant/1 -> Communication Issue (0,1)/1
